simulink model "blance_leg2"  (R2023a)
settings: Solver=VariableStepAuto  StartTime=0.0  StopTime=10  MaxStep=0.0050000000000000001  RelTol=5.0000000000000002e-05  AbsTol=9.9999999999999995e-07
InitFcn:
  | addpath(fileparts(get_param(bdroot,'FileName')));
  | apply_config(bdroot);
model workspace (MAT data in the model file):
  L_length_ref : timeseries (value not decoded)
  L_v_ref : timeseries (value not decoded)
  R_length_ref : timeseries (value not decoded)
  R_v_ref : timeseries (value not decoded)
  runScenario_cfg_override = []
  wheel_speed_compensation = 1
values from neighbouring files (symbols this model uses):
  K = cachedK    [configured_lqr_gain.m]    (also in get_k_length.m = lqr(A,B,Q,R); matlab.mat = [-1.73670717704  -0.157075032659  -0.691811333866  -0.787613)
  N = NM + mp*diff(x + L*sin(theta),t,2)    [get_k_length.m]
  s = sin(phi3 - phi2)    [five_bar_geometry_rm.m]
undefined symbols (not defined in the file or in its folder): X, Y, Z
libraries: sm_lib x82, nesl_utility x35, slpidlib x2
(part 3 of 3)

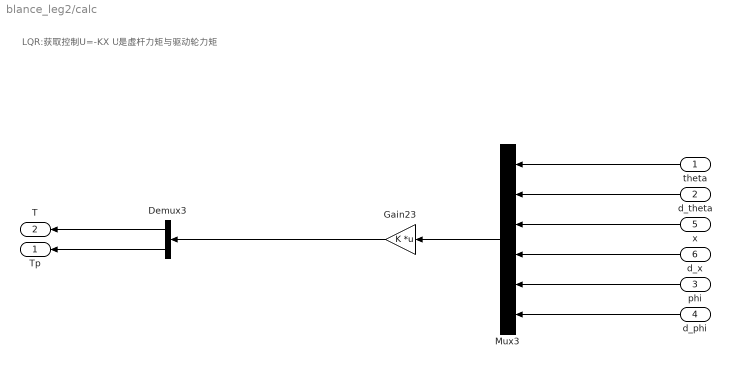
== system blance_leg2/calc ==
  note: LQR:获取控制U=-KX
      | U是虚杆力矩与驱动轮力矩
  theta : Inport
  d_theta : Inport  Port=2
  phi : Inport  Port=3
  d_phi : Inport  Port=4
  x : Inport  Port=5
  d_x : Inport  Port=6
  Demux3 : Demux  Outputs=2
  Gain23 : Gain  Gain=K  Multiplication=Matrix(K*u) (u vector)
  Mux3 : Mux  Inputs=6
  Tp : Outport
  T : Outport  Port=2
  wires:
  Demux3/1 -> T/1
  Demux3/2 -> Tp/1
  Mux3/1 -> Gain23/1
  theta/1 -> Mux3/1
  d_theta/1 -> Mux3/2
  x/1 -> Mux3/3
  d_x/1 -> Mux3/4
  phi/1 -> Mux3/5
  d_phi/1 -> Mux3/6
  Gain23/1 -> Demux3/1

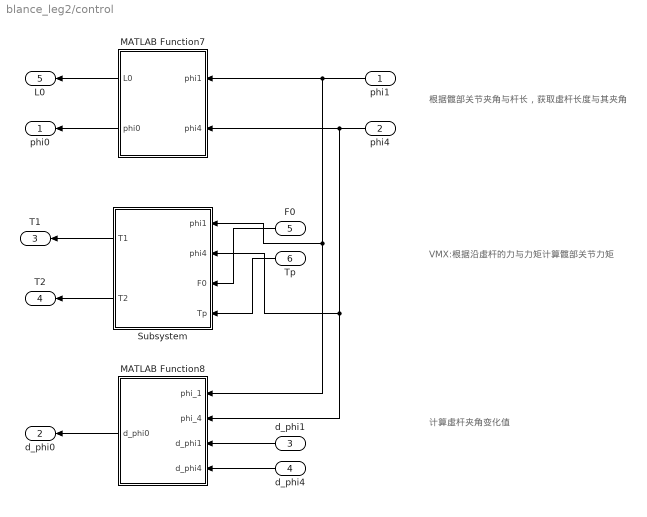
== system blance_leg2/control ==
  note: 计算虚杆夹角变化值
  note: VMX:根据沿虚杆的力与力矩计算髋部关节力矩
  note: 根据髋部关节夹角与杆长，获取虚杆长度与其夹角
  phi1 : Inport
  phi4 : Inport  Port=2
  d_phi1 : Inport  Port=3
  d_phi4 : Inport  Port=4
  F0 : Inport  Port=5
  Tp : Inport  Port=6
  MATLAB Function7 : MATLAB Function  TreatAsAtomicUnit=on
  MATLAB Function8 : MATLAB Function  TreatAsAtomicUnit=on
  Subsystem : Subsystem
  phi0 : Outport
  d_phi0 : Outport  Port=2
  T1 : Outport  Port=3
  T2 : Outport  Port=4
  L0 : Outport  Port=5
  wires:
  MATLAB Function7/2(phi0) -> phi0/1
  MATLAB Function8/1(d_phi0) -> d_phi0/1
  d_phi4/1 -> MATLAB Function8/4(d_phi4)
  d_phi1/1 -> MATLAB Function8/3(d_phi1)
  MATLAB Function7/1(L0) -> L0/1
  phi4/1 -> MATLAB Function7/2(phi4), Subsystem/2(phi4), MATLAB Function8/2(phi_4)
  phi1/1 -> MATLAB Function7/1(phi1), MATLAB Function8/1(phi_1), Subsystem/1(phi1)
  F0/1 -> Subsystem/3(F0)
  Tp/1 -> Subsystem/4(Tp)
  Subsystem/1(T1) -> T1/1
  Subsystem/2(T2) -> T2/1

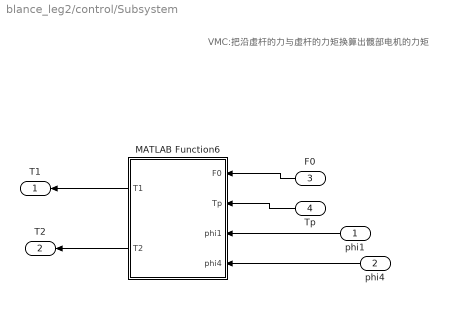
== system blance_leg2/control/Subsystem ==
  note: VMC:把沿虚杆的力与虚杆的力矩换算出髋部电机的力矩
  phi1 : Inport
  phi4 : Inport  Port=2
  F0 : Inport  Port=3
  Tp : Inport  Port=4
  MATLAB Function6 : MATLAB Function  TreatAsAtomicUnit=on
  T1 : Outport
  T2 : Outport  Port=2
  wires:
  phi1/1 -> MATLAB Function6/3(phi1)
  phi4/1 -> MATLAB Function6/4(phi4)
  Tp/1 -> MATLAB Function6/2(Tp)
  MATLAB Function6/1(T1) -> T1/1
  F0/1 -> MATLAB Function6/1(F0)
  MATLAB Function6/2(T2) -> T2/1

== matlab function blance_leg2/Right Wheel Carrier Rate ==
  data: phi1 input; omega output; phi4 input; w1 input; w4 input; bodyPitchRate input
function omega = carrier_world_rate(phi1,phi4,w1,w4,bodyPitchRate)
%#codegen
omega=wheel_carrier_rate(phi1,phi4,w1,w4,bodyPitchRate);
end

== matlab function blance_leg2/Left Wheel Carrier Rate ==
  data: phi1 input; omega output; phi4 input; w1 input; w4 input; bodyPitchRate input
function omega = carrier_world_rate(phi1,phi4,w1,w4,bodyPitchRate)
%#codegen
omega=wheel_carrier_rate(phi1,phi4,w1,w4,bodyPitchRate);
end

== matlab function blance_leg2/Subsystem4/MATLAB Function10 ==
  data: L0 output; phi1 input; phi4 input; phi0 output
function [L0,phi0] = fcn(phi1,phi4)
   
    l5=0.08;%AE长度
    l1=0.075;
    l2=0.14;
    l3=0.14;
    l4=0.075;
    
    YD = l4*sin(phi4);
    YB = l1*sin(phi1);
    XD = l5 + l4*cos(phi4);
    XB = l1*cos(phi1); 
    lBD = sqrt((XD - XB)*(XD - XB) + (YD - YB)*(YD - YB));
    A0 = 2*l2*(XD - XB);
    B0 = 2*l2*(YD - YB);
    C0 = l2*l2 + lBD*lBD - l3*l3;
    phi2 = 2*atan2((B0 + sqrt(A0*A0 + B0*B0 - C0*C0)),(A0 + C0));
    XC = l1*cos(phi1) + l2*cos(phi2);
    YC = l1*sin(phi1) + l2*sin(phi2);
    L0 = sqrt((XC - l5/2)*(XC - l5/2) + YC*YC);
    phi0=atan2(YC,(XC-l5/2));
    
end

== matlab function blance_leg2/Subsystem4/MATLAB Function11 ==
  data: d_phi0 output; phi_1 input; phi_4 input; d_phi1 input; d_phi4 input
function d_phi0 = fcn(phi_1,phi_4,d_phi1,d_phi4)
   
    l5=0.08;%AE长度
    l1=0.075;
    l2=0.14;
    l3=0.14;
    l4=0.075;
    
    d_phi0 = (d_phi1*((l1*cos(phi_1) + (2*l2*cos(2*atan(((4*l2^2*(l1*sin(phi_1) - l4*sin(phi_4))^2 - ((l1*sin(phi_1) - l4*sin(phi_4))^2 + (l5 - l1*cos(phi_1) + l4*cos(phi_4))^2 + l2^2 - l3^2)^2 + 4*l2^2*(l5 - l1*cos(phi_1) + l4*cos(phi_4))^2)^(1/2) - 2*l2*(l1*sin(phi_1) - l4*sin(phi_4)))/((l1*sin(phi_1) - l4*sin(phi_4))^2 + (l5 - l1*cos(phi_1) + l4*cos(phi_4))^2 + l2^2 - l3^2 + 2*l2*(l5 - l1*cos(phi_1) + l4*cos(phi_4)))))*(((8*l1*l2^2*cos(phi_1)*(l1*sin(phi_1) - l4*sin(phi_4)) - 2*(2*l1*cos(phi_1)*(l1*sin(phi_1) - l4*sin(phi_4)) + 2*l1*sin(phi_1)*(l5 - l1*cos(phi_1) + l4*cos(phi_4)))*((l1*sin(phi_1) - l4*sin(phi_4))^2 + (l5 - l1*cos(phi_1) + l4*cos(phi_4))^2 + l2^2 - l3^2) + 8*l1*l2^2*sin(phi_1)*(l5 - l1*cos(phi_1) + l4*cos(phi_4)))/(2*(4*l2^2*(l1*sin(phi_1) - l4*sin(phi_4))^2 - ((l1*sin(phi_1) - l4*sin(phi_4))^2 + (l5 - l1*cos(phi_1) + l4*cos(phi_4))^2 + l2^2 - l3^2)^2 + 4*l2^2*(l5 - l1*cos(phi_1) + l4*cos(phi_4))^2)^(1/2)) - 2*l1*l2*cos(phi_1))/((l1*sin(phi_1) - l4*sin(phi_4))^2 + (l5 - l1*cos(phi_1) + l4*cos(phi_4))^2 + l2^2 - l3^2 + 2*l2*(l5 - l1*cos(phi_1) + l4*cos(phi_4))) - (((4*l2^2*(l1*sin(phi_1) - l4*sin(phi_4))^2 - ((l1*sin(phi_1) - l4*sin(phi_4))^2 + (l5 - l1*cos(phi_1) + l4*cos(phi_4))^2 + l2^2 - l3^2)^2 + 4*l2^2*(l5 - l1*cos(phi_1) + l4*cos(phi_4))^2)^(1/2) - 2*l2*(l1*sin(phi_1) - l4*sin(phi_4)))*(2*l1*l2*sin(phi_1) + 2*l1*cos(phi_1)*(l1*sin(phi_1) - l4*sin(phi_4)) + 2*l1*sin(phi_1)*(l5 - l1*cos(phi_1) + l4*cos(phi_4))))/((l1*sin(phi_1) - l4*sin(phi_4))^2 + (l5 - l1*cos(phi_1) + l4*cos(phi_4))^2 + l2^2 - l3^2 + 2*l2*(l5 - l1*cos(phi_1) + l4*cos(phi_4)))^2))/(((4*l2^2*(l1*sin(phi_1) - l4*sin(phi_4))^2 - ((l1*sin(phi_1) - l4*sin(phi_4))^2 + (l5 - l1*cos(phi_1) + l4*cos(phi_4))^2 + l2^2 - l3^2)^2 + 4*l2^2*(l5 - l1*cos(phi_1) + l4*cos(phi_4))^2)^(1/2) - 2*l2*(l1*sin(phi_1) - l4*sin(phi_4)))^2/((l1*sin(phi_1) - l4*sin(phi_4))^2 + (l5 - l1*cos(phi_1) + l4*cos(phi_4))^2 + l2^2 - l3^2 + 2*l2*(l5 - l1*cos(phi_1) + l4*cos(phi_4)))^2 + 1))/(l2*cos(2*atan(((4*l2^2*(l1*sin(phi_1) - l4*sin(phi_4))^2 - ((l1*sin(phi_1) - l4*sin(phi_4))^2 + (l5 - l1*cos(phi_1) + l4*cos(phi_4))^2 + l2^2 - l3^2)^2 + 4*l2^2*(l5 - l1*cos(phi_1) + l4*cos(phi_4))^2)^(1/2) - 2*l2*(l1*sin(phi_1) - l4*sin(phi_4)))/((l1*sin(phi_1) - l4*sin(phi_4))^2 + (l5 - l1*cos(phi_1) + l4*cos(phi_4))^2 + l2^2 - l3^2 + 2*l2*(l5 - l1*cos(phi_1) + l4*cos(phi_4))))) - l5/2 + l1*cos(phi_1)) + ((l2*sin(2*atan(((4*l2^2*(l1*sin(phi_1) - l4*sin(phi_4))^2 - ((l1*sin(phi_1) - l4*sin(phi_4))^2 + (l5 - l1*cos(phi_1) + l4*cos(phi_4))^2 + l2^2 - l3^2)^2 + 4*l2^2*(l5 - l1*cos(phi_1) + l4*cos(phi_4))^2)^(1/2) - 2*l2*(l1*sin(phi_1) - l4*sin(phi_4)))/((l1*sin(phi_1) - l4*sin(phi_4))^2 + (l5 - l1*cos(phi_1) + l4*cos(phi_4))^2 + l2^2 - l3^2 + 2*l2*(l5 - l1*cos(phi_1) + l4*cos(phi_4))))) + l1*sin(phi_1))*(l1*sin(phi_1) + (2*l2*sin(2*atan(((4*l2^2*(l1*sin(phi_1) - l4*sin(phi_4))^2 - ((l1*sin(phi_1) - l4*sin(phi_4))^2 + (l5 - l1*cos(phi_1) + l4*cos(phi_4))^2 + l2^2 - l3^2)^2 + 4*l2^2*(l5 - l1*cos(phi_1) + l4*cos(phi_4))^2)^(1/2) - 2*l2*(l1*sin(phi_1) - l4*sin(phi_4)))/((l1*sin(phi_1) - l4*sin(phi_4))^2 + (l5 - l1*cos(phi_1) + l4*cos(phi_4))^2 + l2^2 - l3^2 + 2*l2*(l5 - l1*cos(phi_1) + l4*cos(phi_4)))))*(((8*l1*l2^2*cos(phi_1)*(l1*sin(phi_1) - l4*sin(phi_4)) - 2*(2*l1*cos(phi_1)*(l1*sin(phi_1) - l4*sin(phi_4)) + 2*l1*sin(phi_1)*(l5 - l1*cos(phi_1) + l4*cos(phi_4)))*((l1*sin(phi_1) - l4*sin(phi_4))^2 + (l5 - l1*cos(phi_1) + l4*cos(phi_4))^2 + l2^2 - l3^2) + 8*l1*l2^2*sin(phi_1)*(l5 - l1*cos(phi_1) + l4*cos(phi_4)))/(2*(4*l2^2*(l1*sin(phi_1) - l4*sin(phi_4))^2 - ((l1*sin(phi_1) - l4*sin(phi_4))^2 + (l5 - l1*cos(phi_1) + l4*cos(phi_4))^2 + l2^2 - l3^2)^2 + 4*l2^2*(l5 - l1*cos(phi_1) + l4*cos(phi_4))^2)^(1/2)) - 2*l1*l2*cos(phi_1))/((l1*sin(phi_1) - l4*sin(phi_4))^2 + (l5 - l1*cos(phi_1) + l4*cos(phi_4))^2 + l2^2 - l3^2 + 2*l2*(l5 - l1*cos(phi_1) + l4*cos(phi_4))) - (((4*l2^2*(l1*sin(phi_1) - l4*sin(phi_4))^2 - ((l1*sin(phi_1) - l4*sin(phi_4))^2 + (l5 - l1*cos(phi_1) + l4*cos(phi_4))^2 + l2^2 - l3^2)^2 + 4*l2^2*(l5 - l1*cos(phi_1) + l4*cos(phi_4))^2)^(1/2) - 2*l2*(l1*sin(phi_1) - l4*sin(phi_4)))*(2*l1*l2*sin(phi_1) + 2*l1*cos(phi_1)*(l1*sin(phi_1) - l4*sin(phi_4)) + 2*l1*sin(phi_1)*(l5 - l1*cos(phi_1) + l4*cos(phi_4))))/((l1*sin(phi_1) - l4*sin(phi_4))^2 + (l5 - l1*cos(phi_1) + l4*cos(phi_4))^2 + l2^2 - l3^2 + 2*l2*(l5 - l1*cos(phi_1) + l4*cos(phi_4)))^2))/(((4*l2^2*(l1*sin(phi_1) - l4*sin(phi_4))^2 - ((l1*sin(phi_1) - l4*sin(phi_4))^2 + (l5 - l1*cos(phi_1) + l4*cos(phi_4))^2 + l2^2 - l3^2)^2 + 4*l2^2*(l5 - l1*cos(phi_1) + l4*cos(phi_4))^2)^(1/2) - 2*l2*(l1*sin(phi_1) - l4*sin(phi_4)))^2/((l1*sin(phi_1) - l4*sin(phi_4))^2 + (l5 - l1*cos(phi_1) + l4*cos(phi_4))^2 + l2^2 - l3^2 + 2*l2*(l5 - l1*cos(phi_1) + l4*cos(phi_4)))^2 + 1)))/(l2*cos(2*atan(((4*l2^2*(l1*sin(phi_1) - l4*sin(phi_4))^2 - ((l1*sin(phi_1) - l4*sin(phi_4))^2 + (l5 - l1*cos(phi_1) + l4*cos(phi_4))^2 + l2^2 - l3^2)^2 + 4*l2^2*(l5 - l1*cos(phi_1) + l4*cos(phi_4))^2)^(1/2) - 2*l2*(l1*sin(phi_1) - l4*sin(phi_4)))/((l1*sin(phi_1) - l4*sin(phi_4))^2 + (l5 - l1*cos(phi_1) + l4*cos(phi_4))^2 + l2^2 - l3^2 + 2*l2*(l5 - l1*cos(phi_1) + l4*cos(phi_4))))) - l5/2 + l1*cos(phi_1))^2))/((l2*sin(2*atan(((4*l2^2*(l1*sin(phi_1) - l4*sin(phi_4))^2 - ((l1*sin(phi_1) - l4*sin(phi_4))^2 + (l5 - l1*cos(phi_1) + l4*cos(phi_4))^2 + l2^2 - l3^2)^2 + 4*l2^2*(l5 - l1*cos(phi_1) + l4*cos(phi_4))^2)^(1/2) - 2*l2*(l1*sin(phi_1) - l4*sin(phi_4)))/((l1*sin(phi_1) - l4*sin(phi_4))^2 + (l5 - l1*cos(phi_1) + l4*cos(phi_4))^2 + l2^2 - l3^2 + 2*l2*(l5 - l1*cos(phi_1) + l4*cos(phi_4))))) + l1*sin(phi_1))^2/(l2*cos(2*atan(((4*l2^2*(l1*sin(phi_1) - l4*sin(phi_4))^2 - ((l1*sin(phi_1) - l4*sin(phi_4))^2 + (l5 - l1*cos(phi_1) + l4*cos(phi_4))^2 + l2^2 - l3^2)^2 + 4*l2^2*(l5 - l1*cos(phi_1) + l4*cos(phi_4))^2)^(1/2) - 2*l2*(l1*sin(phi_1) - l4*sin(phi_4)))/((l1*sin(phi_1) - l4*sin(phi_4))^2 + (l5 - l1*cos(phi_1) + l4*cos(phi_4))^2 + l2^2 - l3^2 + 2*l2*(l5 - l1*cos(phi_1) + l4*cos(phi_4))))) - l5/2 + l1*cos(phi_1))^2 + 1) - (d_phi4*((2*l2*cos(2*atan(((4*l2^2*(l1*sin(phi_1) - l4*sin(phi_4))^2 - ((l1*sin(phi_1) - l4*sin(phi_4))^2 + (l5 - l1*cos(phi_1) + l4*cos(phi_4))^2 + l2^2 - l3^2)^2 + 4*l2^2*(l5 - l1*cos(phi_1) + l4*cos(phi_4))^2)^(1/2) - 2*l2*(l1*sin(phi_1) - l4*sin(phi_4)))/((l1*sin(phi_1) - l4*sin(phi_4))^2 + (l5 - l1*cos(phi_1) + l4*cos(phi_4))^2 + l2^2 - l3^2 + 2*l2*(l5 - l1*cos(phi_1) + l4*cos(phi_4)))))*(((8*l2^2*l4*cos(phi_4)*(l1*sin(phi_1) - l4*sin(phi_4)) - 2*(2*l4*cos(phi_4)*(l1*sin(phi_1) - l4*sin(phi_4)) + 2*l4*sin(phi_4)*(l5 - l1*cos(phi_1) + l4*cos(phi_4)))*((l1*sin(phi_1) - l4*sin(phi_4))^2 + (l5 - l1*cos(phi_1) + l4*cos(phi_4))^2 + l2^2 - l3^2) + 8*l2^2*l4*sin(phi_4)*(l5 - l1*cos(phi_1) + l4*cos(phi_4)))/(2*(4*l2^2*(l1*sin(phi_1) - l4*sin(phi_4))^2 - ((l1*sin(phi_1) - l4*sin(phi_4))^2 + (l5 - l1*cos(phi_1) + l4*cos(phi_4))^2 + l2^2 - l3^2)^2 + 4*l2^2*(l5 - l1*cos(phi_1) + l4*cos(phi_4))^2)^(1/2)) - 2*l2*l4*cos(phi_4))/((l1*sin(phi_1) - l4*sin(phi_4))^2 + (l5 - l1*cos(phi_1) + l4*cos(phi_4))^2 + l2^2 - l3^2 + 2*l2*(l5 - l1*cos(phi_1) + l4*cos(phi_4))) - (((4*l2^2*(l1*sin(phi_1) - l4*sin(phi_4))^2 - ((l1*sin(phi_1) - l4*sin(phi_4))^2 + (l5 - l1*cos(phi_1) + l4*cos(phi_4))^2 + l2^2 - l3^2)^2 + 4*l2^2*(l5 - l1*cos(phi_1) + l4*cos(phi_4))^2)^(1/2) - 2*l2*(l1*sin(phi_1) - l4*sin(phi_4)))*(2*l2*l4*sin(phi_4) + 2*l4*cos(phi_4)*(l1*sin(phi_1) - l4*sin(phi_4)) + 2*l4*sin(phi_4)*(l5 - l1*cos(phi_1) + l4*cos(phi_4))))/((l1*sin(phi_1) - l4*sin(phi_4))^2 + (l5 - l1*cos(phi_1) + l4*cos(phi_4))^2 + l2^2 - l3^2 + 2*l2*(l5 - l1*cos(phi_1) + l4*cos(phi_4)))^2))/((((4*l2^2*(l1*sin(phi_1) - l4*sin(phi_4))^2 - ((l1*sin(phi_1) - l4*sin(phi_4))^2 + (l5 - l1*cos(phi_1) + l4*cos(phi_4))^2 + l2^2 - l3^2)^2 + 4*l2^2*(l5 - l1*cos(phi_1) + l4*cos(phi_4))^2)^(1/2) - 2*l2*(l1*sin(phi_1) - l4*sin(phi_4)))^2/((l1*sin(phi_1) - l4*sin(phi_4))^2 + (l5 - l1*cos(phi_1) + l4*cos(phi_4))^2 + l2^2 - l3^2 + 2*l2*(l5 - l1*cos(phi_1) + l4*cos(phi_4)))^2 + 1)*(l2*cos(2*atan(((4*l2^2*(l1*sin(phi_1) - l4*sin(phi_4))^2 - ((l1*sin(phi_1) - l4*sin(phi_4))^2 + (l5 - l1*cos(phi_1) + l4*cos(phi_4))^2 + l2^2 - l3^2)^2 + 4*l2^2*(l5 - l1*cos(phi_1) + l4*cos(phi_4))^2)^(1/2) - 2*l2*(l1*sin(phi_1) - l4*sin(phi_4)))/((l1*sin(phi_1) - l4*sin(phi_4))^2 + (l5 - l1*cos(phi_1) + l4*cos(phi_4))^2 + l2^2 - l3^2 + 2*l2*(l5 - l1*cos(phi_1) + l4*cos(phi_4))))) - l5/2 + l1*cos(phi_1))) + (2*l2*sin(2*atan(((4*l2^2*(l1*sin(phi_1) - l4*sin(phi_4))^2 - ((l1*sin(phi_1) - l4*sin(phi_4))^2 + (l5 - l1*cos(phi_1) + l4*cos(phi_4))^2 + l2^2 - l3^2)^2 + 4*l2^2*(l5 - l1*cos(phi_1) + l4*cos(phi_4))^2)^(1/2) - 2*l2*(l1*sin(phi_1) - l4*sin(phi_4)))/((l1*sin(phi_1) - l4*sin(phi_4))^2 + (l5 - l1*cos(phi_1) + l4*cos(phi_4))^2 + l2^2 - l3^2 + 2*l2*(l5 - l1*cos(phi_1) + l4*cos(phi_4)))))*(l2*sin(2*atan(((4*l2^2*(l1*sin(phi_1) - l4*sin(phi_4))^2 - ((l1*sin(phi_1) - l4*sin(phi_4))^2 + (l5 - l1*cos(phi_1) + l4*cos(phi_4))^2 + l2^2 - l3^2)^2 + 4*l2^2*(l5 - l1*cos(phi_1) + l4*cos(phi_4))^2)^(1/2) - 2*l2*(l1*sin(phi_1) - l4*sin(phi_4)))/((l1*sin(phi_1) - l4*sin(phi_4))^2 + (l5 - l1*cos(phi_1) + l4*cos(phi_4))^2 + l2^2 - l3^2 + 2*l2*(l5 - l1*cos(phi_1) + l4*cos(phi_4))))) + l1*sin(phi_1))*(((8*l2^2*l4*cos(phi_4)*(l1*sin(phi_1) - l4*sin(phi_4)) - 2*(2*l4*cos(phi_4)*(l1*sin(phi_1) - l4*sin(phi_4)) + 2*l4*sin(phi_4)*(l5 - l1*cos(phi_1) + l4*cos(phi_4)))*((l1*sin(phi_1) - l4*sin(phi_4))^2 + (l5 - l1*cos(phi_1) + l4*cos(phi_4))^2 + l2^2 - l3^2) + 8*l2^2*l4*sin(phi_4)*(l5 - l1*cos(phi_1) + l4*cos(phi_4)))/(2*(4*l2^2*(l1*sin(phi_1) - l4*sin(phi_4))^2 - ((l1*sin(phi_1) - l4*sin(phi_4))^2 + (l5 - l1*cos(phi_1) + l4*cos(phi_4))^2 + l2^2 - l3^2)^2 + 4*l2^2*(l5 - l1*cos(phi_1) + l4*cos(phi_4))^2)^(1/2)) - 2*l2*l4*cos(phi_4))/((l1*sin(phi_1) - l4*sin(phi_4))^2 + (l5 - l1*cos(phi_1) + l4*cos(phi_4))^2 + l2^2 - l3^2 + 2*l2*(l5 - l1*cos(phi_1) + l4*cos(phi_4))) - (((4*l2^2*(l1*sin(phi_1) - l4*sin(phi_4))^2 - ((l1*sin(phi_1) - l4*sin(phi_4))^2 + (l5 - l1*cos(phi_1) + l4*cos(phi_4))^2 + l2^2 - l3^2)^2 + 4*l2^2*(l5 - l1*cos(phi_1) + l4*cos(phi_4))^2)^(1/2) - 2*l2*(l1*sin(phi_1) - l4*sin(phi_4)))*(2*l2*l4*sin(phi_4) + 2*l4*cos(phi_4)*(l1*sin(phi_1) - l4*sin(phi_4)) + 2*l4*sin(phi_4)*(l5 - l1*cos(phi_1) + l4*cos(phi_4))))/((l1*sin(phi_1) - l4*sin(phi_4))^2 + (l5 - l1*cos(phi_1) + l4*cos(phi_4))^2 + l2^2 - l3^2 + 2*l2*(l5 - l1*cos(phi_1) + l4*cos(phi_4)))^2))/((((4*l2^2*(l1*sin(phi_1) - l4*sin(phi_4))^2 - ((l1*sin(phi_1) - l4*sin(phi_4))^2 + (l5 - l1*cos(phi_1) + l4*cos(phi_4))^2 + l2^2 - l3^2)^2 + 4*l2^2*(l5 - l1*cos(phi_1) + l4*cos(phi_4))^2)^(1/2) - 2*l2*(l1*sin(phi_1) - l4*sin(phi_4)))^2/((l1*sin(phi_1) - l4*sin(phi_4))^2 + (l5 - l1*cos(phi_1) + l4*cos(phi_4))^2 + l2^2 - l3^2 + 2*l2*(l5 - l1*cos(phi_1) + l4*cos(phi_4)))^2 + 1)*(l2*cos(2*atan(((4*l2^2*(l1*sin(phi_1) - l4*sin(phi_4))^2 - ((l1*sin(phi_1) - l4*sin(phi_4))^2 + (l5 - l1*cos(phi_1) + l4*cos(phi_4))^2 + l2^2 - l3^2)^2 + 4*l2^2*(l5 - l1*cos(phi_1) + l4*cos(phi_4))^2)^(1/2) - 2*l2*(l1*sin(phi_1) - l4*sin(phi_4)))/((l1*sin(phi_1) - l4*sin(phi_4))^2 + (l5 - l1*cos(phi_1) + l4*cos(phi_4))^2 + l2^2 - l3^2 + 2*l2*(l5 - l1*cos(phi_1) + l4*cos(phi_4))))) - l5/2 + l1*cos(phi_1))^2)))/((l2*sin(2*atan(((4*l2^2*(l1*sin(phi_1) - l4*sin(phi_4))^2 - ((l1*sin(phi_1) - l4*sin(phi_4))^2 + (l5 - l1*cos(phi_1) + l4*cos(phi_4))^2 + l2^2 - l3^2)^2 + 4*l2^2*(l5 - l1*cos(phi_1) + l4*cos(phi_4))^2)^(1/2) - 2*l2*(l1*sin(phi_1) - l4*sin(phi_4)))/((l1*sin(phi_1) - l4*sin(phi_4))^2 + (l5 - l1*cos(phi_1) + l4*cos(phi_4))^2 + l2^2 - l3^2 + 2*l2*(l5 - l1*cos(phi_1) + l4*cos(phi_4))))) + l1*sin(phi_1))^2/(l2*cos(2*atan(((4*l2^2*(l1*sin(phi_1) - l4*sin(phi_4))^2 - ((l1*sin(phi_1) - l4*sin(phi_4))^2 + (l5 - l1*cos(phi_1) + l4*cos(phi_4))^2 + l2^2 - l3^2)^2 + 4*l2^2*(l5 - l1*cos(phi_1) + l4*cos(phi_4))^2)^(1/2) - 2*l2*(l1*sin(phi_1) - l4*sin(phi_4)))/((l1*sin(phi_1) - l4*sin(phi_4))^2 + (l5 - l1*cos(phi_1) + l4*cos(phi_4))^2 + l2^2 - l3^2 + 2*l2*(l5 - l1*cos(phi_1) + l4*cos(phi_4))))) - l5/2 + l1*cos(phi_1))^2 + 1);
end
    % syms phi_0 phi_1 phi_2 phi_4 l1 l2 l3 l4 l5 L0 d_phi1 d_phi4
    % 
    % XD=l5+l4*cos(phi_4);
    % YD=l4*sin(phi_4);
    % XB=l1*cos(phi_1);
    % YB=l1*sin(phi_1);
    % A0=2*l2*(XD-XB);
    % B0=2*l2*(YD-YB);
    % lBD=sqrt((XD-XB)^2+(YD-YB)^2);
    % C0=l2^2+lBD^2-l3^2;
    % phi_2=2*atan((B0+sqrt(A0^2+B0^2-C0^2))/(A0+C0));
    % XC=XB+l2*cos(phi_2);
    % YC=YB+l2*sin(phi_2);
    % L0=sqrt((XC-l5/2)^2+YC^2);
    % phi_0=atan(YC/(XC-l5/2));
    % 
    % J=jacobian([L0;phi_0],[phi_1;phi_4]);
    % phi0_dot = J(2,1)*d_phi1 +J(2,2)*d_phi4

    % jacobian函数无法在simulink中使用，故直接使用jacobian函数的最终结果

== matlab function blance_leg2/control/Subsystem/MATLAB Function6 ==
  data: F0 input; T1 output; Tp input; phi1 input; phi4 input; T2 output
function [T1,T2] = VMC_calc(F0,Tp,phi1,phi4)

    l5=0.08;%AE长度
    l1=0.075;
    l2=0.14;
    l3=0.14;
    l4=0.075;

YD = l4*sin(phi4);
YB = l1*sin(phi1);
XD = l5 + l4*cos(phi4);
XB = l1*cos(phi1); 
lBD = sqrt((XD - XB)*(XD - XB) + (YD - YB)*(YD - YB));
A0 = 2*l2*(XD - XB);
B0 = 2*l2*(YD - YB);
C0 = l2*l2 + lBD*lBD - l3*l3;
phi2 = 2*atan2((B0 + sqrt(A0*A0 + B0*B0 - C0*C0)),A0 + C0);
phi3 = atan2(YB-YD+l2*sin(phi2),XB-XD+l2*cos(phi2));
XC = l1*cos(phi1) + l2*cos(phi2);
YC = l1*sin(phi1) + l2*sin(phi2);
L0 = sqrt((XC - l5/2)*(XC - l5/2) + YC*YC);
phi0 = atan2(YC,XC - l5/2);
j11 = (l1*sin(phi0-phi3)*sin(phi1-phi2))/sin(phi3-phi2);
j12 = (l1*cos(phi0-phi3)*sin(phi1-phi2))/(L0*sin(phi3-phi2));
j21 = (l4*sin(phi0-phi2)*sin(phi3-phi4))/sin(phi3-phi2);
j22 = (l4*cos(phi0-phi2)*sin(phi3-phi4))/(L0*sin(phi3-phi2));
J = [j11 j12; j21 j22];
F = [F0;Tp];
T = J * F;
T1 = T(1,1);
T2 = T(2,1);

end

== matlab function blance_leg2/control/MATLAB Function7 ==
  data: L0 output; phi1 input; phi4 input; phi0 output
function [L0,phi0] = fcn(phi1,phi4)
  
    l5=0.08;%AE长度
    l1=0.075;
    l2=0.14;
    l3=0.14;
    l4=0.075;
    
    YD = l4*sin(phi4);
    YB = l1*sin(phi1);
    XD = l5 + l4*cos(phi4);
    XB = l1*cos(phi1); 
    lBD = sqrt((XD - XB)*(XD - XB) + (YD - YB)*(YD - YB));
    A0 = 2*l2*(XD - XB);
    B0 = 2*l2*(YD - YB);
    C0 = l2*l2 + lBD*lBD - l3*l3;
    phi2 = 2*atan2((B0 + sqrt(A0*A0 + B0*B0 - C0*C0)),(A0 + C0));
    XC = l1*cos(phi1) + l2*cos(phi2);
    YC = l1*sin(phi1) + l2*sin(phi2);
    L0 = sqrt((XC - l5/2)*(XC - l5/2) + YC*YC);
    phi0=atan2(YC,(XC-l5/2));
end

== matlab function blance_leg2/control/MATLAB Function8 ==
  data: d_phi0 output; phi_1 input; phi_4 input; d_phi1 input; d_phi4 input
% 计算虚杆夹角变化值
function d_phi0 = fcn(phi_1,phi_4,d_phi1,d_phi4)
   
    l5=0.08;%AE长度
    l1=0.075;
    l2=0.14;
    l3=0.14;
    l4=0.075;
    
    d_phi0 = (d_phi1*((l1*cos(phi_1) + (2*l2*cos(2*atan(((4*l2^2*(l1*sin(phi_1) - l4*sin(phi_4))^2 - ((l1*sin(phi_1) - l4*sin(phi_4))^2 + (l5 - l1*cos(phi_1) + l4*cos(phi_4))^2 + l2^2 - l3^2)^2 + 4*l2^2*(l5 - l1*cos(phi_1) + l4*cos(phi_4))^2)^(1/2) - 2*l2*(l1*sin(phi_1) - l4*sin(phi_4)))/((l1*sin(phi_1) - l4*sin(phi_4))^2 + (l5 - l1*cos(phi_1) + l4*cos(phi_4))^2 + l2^2 - l3^2 + 2*l2*(l5 - l1*cos(phi_1) + l4*cos(phi_4)))))*(((8*l1*l2^2*cos(phi_1)*(l1*sin(phi_1) - l4*sin(phi_4)) - 2*(2*l1*cos(phi_1)*(l1*sin(phi_1) - l4*sin(phi_4)) + 2*l1*sin(phi_1)*(l5 - l1*cos(phi_1) + l4*cos(phi_4)))*((l1*sin(phi_1) - l4*sin(phi_4))^2 + (l5 - l1*cos(phi_1) + l4*cos(phi_4))^2 + l2^2 - l3^2) + 8*l1*l2^2*sin(phi_1)*(l5 - l1*cos(phi_1) + l4*cos(phi_4)))/(2*(4*l2^2*(l1*sin(phi_1) - l4*sin(phi_4))^2 - ((l1*sin(phi_1) - l4*sin(phi_4))^2 + (l5 - l1*cos(phi_1) + l4*cos(phi_4))^2 + l2^2 - l3^2)^2 + 4*l2^2*(l5 - l1*cos(phi_1) + l4*cos(phi_4))^2)^(1/2)) - 2*l1*l2*cos(phi_1))/((l1*sin(phi_1) - l4*sin(phi_4))^2 + (l5 - l1*cos(phi_1) + l4*cos(phi_4))^2 + l2^2 - l3^2 + 2*l2*(l5 - l1*cos(phi_1) + l4*cos(phi_4))) - (((4*l2^2*(l1*sin(phi_1) - l4*sin(phi_4))^2 - ((l1*sin(phi_1) - l4*sin(phi_4))^2 + (l5 - l1*cos(phi_1) + l4*cos(phi_4))^2 + l2^2 - l3^2)^2 + 4*l2^2*(l5 - l1*cos(phi_1) + l4*cos(phi_4))^2)^(1/2) - 2*l2*(l1*sin(phi_1) - l4*sin(phi_4)))*(2*l1*l2*sin(phi_1) + 2*l1*cos(phi_1)*(l1*sin(phi_1) - l4*sin(phi_4)) + 2*l1*sin(phi_1)*(l5 - l1*cos(phi_1) + l4*cos(phi_4))))/((l1*sin(phi_1) - l4*sin(phi_4))^2 + (l5 - l1*cos(phi_1) + l4*cos(phi_4))^2 + l2^2 - l3^2 + 2*l2*(l5 - l1*cos(phi_1) + l4*cos(phi_4)))^2))/(((4*l2^2*(l1*sin(phi_1) - l4*sin(phi_4))^2 - ((l1*sin(phi_1) - l4*sin(phi_4))^2 + (l5 - l1*cos(phi_1) + l4*cos(phi_4))^2 + l2^2 - l3^2)^2 + 4*l2^2*(l5 - l1*cos(phi_1) + l4*cos(phi_4))^2)^(1/2) - 2*l2*(l1*sin(phi_1) - l4*sin(phi_4)))^2/((l1*sin(phi_1) - l4*sin(phi_4))^2 + (l5 - l1*cos(phi_1) + l4*cos(phi_4))^2 + l2^2 - l3^2 + 2*l2*(l5 - l1*cos(phi_1) + l4*cos(phi_4)))^2 + 1))/(l2*cos(2*atan(((4*l2^2*(l1*sin(phi_1) - l4*sin(phi_4))^2 - ((l1*sin(phi_1) - l4*sin(phi_4))^2 + (l5 - l1*cos(phi_1) + l4*cos(phi_4))^2 + l2^2 - l3^2)^2 + 4*l2^2*(l5 - l1*cos(phi_1) + l4*cos(phi_4))^2)^(1/2) - 2*l2*(l1*sin(phi_1) - l4*sin(phi_4)))/((l1*sin(phi_1) - l4*sin(phi_4))^2 + (l5 - l1*cos(phi_1) + l4*cos(phi_4))^2 + l2^2 - l3^2 + 2*l2*(l5 - l1*cos(phi_1) + l4*cos(phi_4))))) - l5/2 + l1*cos(phi_1)) + ((l2*sin(2*atan(((4*l2^2*(l1*sin(phi_1) - l4*sin(phi_4))^2 - ((l1*sin(phi_1) - l4*sin(phi_4))^2 + (l5 - l1*cos(phi_1) + l4*cos(phi_4))^2 + l2^2 - l3^2)^2 + 4*l2^2*(l5 - l1*cos(phi_1) + l4*cos(phi_4))^2)^(1/2) - 2*l2*(l1*sin(phi_1) - l4*sin(phi_4)))/((l1*sin(phi_1) - l4*sin(phi_4))^2 + (l5 - l1*cos(phi_1) + l4*cos(phi_4))^2 + l2^2 - l3^2 + 2*l2*(l5 - l1*cos(phi_1) + l4*cos(phi_4))))) + l1*sin(phi_1))*(l1*sin(phi_1) + (2*l2*sin(2*atan(((4*l2^2*(l1*sin(phi_1) - l4*sin(phi_4))^2 - ((l1*sin(phi_1) - l4*sin(phi_4))^2 + (l5 - l1*cos(phi_1) + l4*cos(phi_4))^2 + l2^2 - l3^2)^2 + 4*l2^2*(l5 - l1*cos(phi_1) + l4*cos(phi_4))^2)^(1/2) - 2*l2*(l1*sin(phi_1) - l4*sin(phi_4)))/((l1*sin(phi_1) - l4*sin(phi_4))^2 + (l5 - l1*cos(phi_1) + l4*cos(phi_4))^2 + l2^2 - l3^2 + 2*l2*(l5 - l1*cos(phi_1) + l4*cos(phi_4)))))*(((8*l1*l2^2*cos(phi_1)*(l1*sin(phi_1) - l4*sin(phi_4)) - 2*(2*l1*cos(phi_1)*(l1*sin(phi_1) - l4*sin(phi_4)) + 2*l1*sin(phi_1)*(l5 - l1*cos(phi_1) + l4*cos(phi_4)))*((l1*sin(phi_1) - l4*sin(phi_4))^2 + (l5 - l1*cos(phi_1) + l4*cos(phi_4))^2 + l2^2 - l3^2) + 8*l1*l2^2*sin(phi_1)*(l5 - l1*cos(phi_1) + l4*cos(phi_4)))/(2*(4*l2^2*(l1*sin(phi_1) - l4*sin(phi_4))^2 - ((l1*sin(phi_1) - l4*sin(phi_4))^2 + (l5 - l1*cos(phi_1) + l4*cos(phi_4))^2 + l2^2 - l3^2)^2 + 4*l2^2*(l5 - l1*cos(phi_1) + l4*cos(phi_4))^2)^(1/2)) - 2*l1*l2*cos(phi_1))/((l1*sin(phi_1) - l4*sin(phi_4))^2 + (l5 - l1*cos(phi_1) + l4*cos(phi_4))^2 + l2^2 - l3^2 + 2*l2*(l5 - l1*cos(phi_1) + l4*cos(phi_4))) - (((4*l2^2*(l1*sin(phi_1) - l4*sin(phi_4))^2 - ((l1*sin(phi_1) - l4*sin(phi_4))^2 + (l5 - l1*cos(phi_1) + l4*cos(phi_4))^2 + l2^2 - l3^2)^2 + 4*l2^2*(l5 - l1*cos(phi_1) + l4*cos(phi_4))^2)^(1/2) - 2*l2*(l1*sin(phi_1) - l4*sin(phi_4)))*(2*l1*l2*sin(phi_1) + 2*l1*cos(phi_1)*(l1*sin(phi_1) - l4*sin(phi_4)) + 2*l1*sin(phi_1)*(l5 - l1*cos(phi_1) + l4*cos(phi_4))))/((l1*sin(phi_1) - l4*sin(phi_4))^2 + (l5 - l1*cos(phi_1) + l4*cos(phi_4))^2 + l2^2 - l3^2 + 2*l2*(l5 - l1*cos(phi_1) + l4*cos(phi_4)))^2))/(((4*l2^2*(l1*sin(phi_1) - l4*sin(phi_4))^2 - ((l1*sin(phi_1) - l4*sin(phi_4))^2 + (l5 - l1*cos(phi_1) + l4*cos(phi_4))^2 + l2^2 - l3^2)^2 + 4*l2^2*(l5 - l1*cos(phi_1) + l4*cos(phi_4))^2)^(1/2) - 2*l2*(l1*sin(phi_1) - l4*sin(phi_4)))^2/((l1*sin(phi_1) - l4*sin(phi_4))^2 + (l5 - l1*cos(phi_1) + l4*cos(phi_4))^2 + l2^2 - l3^2 + 2*l2*(l5 - l1*cos(phi_1) + l4*cos(phi_4)))^2 + 1)))/(l2*cos(2*atan(((4*l2^2*(l1*sin(phi_1) - l4*sin(phi_4))^2 - ((l1*sin(phi_1) - l4*sin(phi_4))^2 + (l5 - l1*cos(phi_1) + l4*cos(phi_4))^2 + l2^2 - l3^2)^2 + 4*l2^2*(l5 - l1*cos(phi_1) + l4*cos(phi_4))^2)^(1/2) - 2*l2*(l1*sin(phi_1) - l4*sin(phi_4)))/((l1*sin(phi_1) - l4*sin(phi_4))^2 + (l5 - l1*cos(phi_1) + l4*cos(phi_4))^2 + l2^2 - l3^2 + 2*l2*(l5 - l1*cos(phi_1) + l4*cos(phi_4))))) - l5/2 + l1*cos(phi_1))^2))/((l2*sin(2*atan(((4*l2^2*(l1*sin(phi_1) - l4*sin(phi_4))^2 - ((l1*sin(phi_1) - l4*sin(phi_4))^2 + (l5 - l1*cos(phi_1) + l4*cos(phi_4))^2 + l2^2 - l3^2)^2 + 4*l2^2*(l5 - l1*cos(phi_1) + l4*cos(phi_4))^2)^(1/2) - 2*l2*(l1*sin(phi_1) - l4*sin(phi_4)))/((l1*sin(phi_1) - l4*sin(phi_4))^2 + (l5 - l1*cos(phi_1) + l4*cos(phi_4))^2 + l2^2 - l3^2 + 2*l2*(l5 - l1*cos(phi_1) + l4*cos(phi_4))))) + l1*sin(phi_1))^2/(l2*cos(2*atan(((4*l2^2*(l1*sin(phi_1) - l4*sin(phi_4))^2 - ((l1*sin(phi_1) - l4*sin(phi_4))^2 + (l5 - l1*cos(phi_1) + l4*cos(phi_4))^2 + l2^2 - l3^2)^2 + 4*l2^2*(l5 - l1*cos(phi_1) + l4*cos(phi_4))^2)^(1/2) - 2*l2*(l1*sin(phi_1) - l4*sin(phi_4)))/((l1*sin(phi_1) - l4*sin(phi_4))^2 + (l5 - l1*cos(phi_1) + l4*cos(phi_4))^2 + l2^2 - l3^2 + 2*l2*(l5 - l1*cos(phi_1) + l4*cos(phi_4))))) - l5/2 + l1*cos(phi_1))^2 + 1) - (d_phi4*((2*l2*cos(2*atan(((4*l2^2*(l1*sin(phi_1) - l4*sin(phi_4))^2 - ((l1*sin(phi_1) - l4*sin(phi_4))^2 + (l5 - l1*cos(phi_1) + l4*cos(phi_4))^2 + l2^2 - l3^2)^2 + 4*l2^2*(l5 - l1*cos(phi_1) + l4*cos(phi_4))^2)^(1/2) - 2*l2*(l1*sin(phi_1) - l4*sin(phi_4)))/((l1*sin(phi_1) - l4*sin(phi_4))^2 + (l5 - l1*cos(phi_1) + l4*cos(phi_4))^2 + l2^2 - l3^2 + 2*l2*(l5 - l1*cos(phi_1) + l4*cos(phi_4)))))*(((8*l2^2*l4*cos(phi_4)*(l1*sin(phi_1) - l4*sin(phi_4)) - 2*(2*l4*cos(phi_4)*(l1*sin(phi_1) - l4*sin(phi_4)) + 2*l4*sin(phi_4)*(l5 - l1*cos(phi_1) + l4*cos(phi_4)))*((l1*sin(phi_1) - l4*sin(phi_4))^2 + (l5 - l1*cos(phi_1) + l4*cos(phi_4))^2 + l2^2 - l3^2) + 8*l2^2*l4*sin(phi_4)*(l5 - l1*cos(phi_1) + l4*cos(phi_4)))/(2*(4*l2^2*(l1*sin(phi_1) - l4*sin(phi_4))^2 - ((l1*sin(phi_1) - l4*sin(phi_4))^2 + (l5 - l1*cos(phi_1) + l4*cos(phi_4))^2 + l2^2 - l3^2)^2 + 4*l2^2*(l5 - l1*cos(phi_1) + l4*cos(phi_4))^2)^(1/2)) - 2*l2*l4*cos(phi_4))/((l1*sin(phi_1) - l4*sin(phi_4))^2 + (l5 - l1*cos(phi_1) + l4*cos(phi_4))^2 + l2^2 - l3^2 + 2*l2*(l5 - l1*cos(phi_1) + l4*cos(phi_4))) - (((4*l2^2*(l1*sin(phi_1) - l4*sin(phi_4))^2 - ((l1*sin(phi_1) - l4*sin(phi_4))^2 + (l5 - l1*cos(phi_1) + l4*cos(phi_4))^2 + l2^2 - l3^2)^2 + 4*l2^2*(l5 - l1*cos(phi_1) + l4*cos(phi_4))^2)^(1/2) - 2*l2*(l1*sin(phi_1) - l4*sin(phi_4)))*(2*l2*l4*sin(phi_4) + 2*l4*cos(phi_4)*(l1*sin(phi_1) - l4*sin(phi_4)) + 2*l4*sin(phi_4)*(l5 - l1*cos(phi_1) + l4*cos(phi_4))))/((l1*sin(phi_1) - l4*sin(phi_4))^2 + (l5 - l1*cos(phi_1) + l4*cos(phi_4))^2 + l2^2 - l3^2 + 2*l2*(l5 - l1*cos(phi_1) + l4*cos(phi_4)))^2))/((((4*l2^2*(l1*sin(phi_1) - l4*sin(phi_4))^2 - ((l1*sin(phi_1) - l4*sin(phi_4))^2 + (l5 - l1*cos(phi_1) + l4*cos(phi_4))^2 + l2^2 - l3^2)^2 + 4*l2^2*(l5 - l1*cos(phi_1) + l4*cos(phi_4))^2)^(1/2) - 2*l2*(l1*sin(phi_1) - l4*sin(phi_4)))^2/((l1*sin(phi_1) - l4*sin(phi_4))^2 + (l5 - l1*cos(phi_1) + l4*cos(phi_4))^2 + l2^2 - l3^2 + 2*l2*(l5 - l1*cos(phi_1) + l4*cos(phi_4)))^2 + 1)*(l2*cos(2*atan(((4*l2^2*(l1*sin(phi_1) - l4*sin(phi_4))^2 - ((l1*sin(phi_1) - l4*sin(phi_4))^2 + (l5 - l1*cos(phi_1) + l4*cos(phi_4))^2 + l2^2 - l3^2)^2 + 4*l2^2*(l5 - l1*cos(phi_1) + l4*cos(phi_4))^2)^(1/2) - 2*l2*(l1*sin(phi_1) - l4*sin(phi_4)))/((l1*sin(phi_1) - l4*sin(phi_4))^2 + (l5 - l1*cos(phi_1) + l4*cos(phi_4))^2 + l2^2 - l3^2 + 2*l2*(l5 - l1*cos(phi_1) + l4*cos(phi_4))))) - l5/2 + l1*cos(phi_1))) + (2*l2*sin(2*atan(((4*l2^2*(l1*sin(phi_1) - l4*sin(phi_4))^2 - ((l1*sin(phi_1) - l4*sin(phi_4))^2 + (l5 - l1*cos(phi_1) + l4*cos(phi_4))^2 + l2^2 - l3^2)^2 + 4*l2^2*(l5 - l1*cos(phi_1) + l4*cos(phi_4))^2)^(1/2) - 2*l2*(l1*sin(phi_1) - l4*sin(phi_4)))/((l1*sin(phi_1) - l4*sin(phi_4))^2 + (l5 - l1*cos(phi_1) + l4*cos(phi_4))^2 + l2^2 - l3^2 + 2*l2*(l5 - l1*cos(phi_1) + l4*cos(phi_4)))))*(l2*sin(2*atan(((4*l2^2*(l1*sin(phi_1) - l4*sin(phi_4))^2 - ((l1*sin(phi_1) - l4*sin(phi_4))^2 + (l5 - l1*cos(phi_1) + l4*cos(phi_4))^2 + l2^2 - l3^2)^2 + 4*l2^2*(l5 - l1*cos(phi_1) + l4*cos(phi_4))^2)^(1/2) - 2*l2*(l1*sin(phi_1) - l4*sin(phi_4)))/((l1*sin(phi_1) - l4*sin(phi_4))^2 + (l5 - l1*cos(phi_1) + l4*cos(phi_4))^2 + l2^2 - l3^2 + 2*l2*(l5 - l1*cos(phi_1) + l4*cos(phi_4))))) + l1*sin(phi_1))*(((8*l2^2*l4*cos(phi_4)*(l1*sin(phi_1) - l4*sin(phi_4)) - 2*(2*l4*cos(phi_4)*(l1*sin(phi_1) - l4*sin(phi_4)) + 2*l4*sin(phi_4)*(l5 - l1*cos(phi_1) + l4*cos(phi_4)))*((l1*sin(phi_1) - l4*sin(phi_4))^2 + (l5 - l1*cos(phi_1) + l4*cos(phi_4))^2 + l2^2 - l3^2) + 8*l2^2*l4*sin(phi_4)*(l5 - l1*cos(phi_1) + l4*cos(phi_4)))/(2*(4*l2^2*(l1*sin(phi_1) - l4*sin(phi_4))^2 - ((l1*sin(phi_1) - l4*sin(phi_4))^2 + (l5 - l1*cos(phi_1) + l4*cos(phi_4))^2 + l2^2 - l3^2)^2 + 4*l2^2*(l5 - l1*cos(phi_1) + l4*cos(phi_4))^2)^(1/2)) - 2*l2*l4*cos(phi_4))/((l1*sin(phi_1) - l4*sin(phi_4))^2 + (l5 - l1*cos(phi_1) + l4*cos(phi_4))^2 + l2^2 - l3^2 + 2*l2*(l5 - l1*cos(phi_1) + l4*cos(phi_4))) - (((4*l2^2*(l1*sin(phi_1) - l4*sin(phi_4))^2 - ((l1*sin(phi_1) - l4*sin(phi_4))^2 + (l5 - l1*cos(phi_1) + l4*cos(phi_4))^2 + l2^2 - l3^2)^2 + 4*l2^2*(l5 - l1*cos(phi_1) + l4*cos(phi_4))^2)^(1/2) - 2*l2*(l1*sin(phi_1) - l4*sin(phi_4)))*(2*l2*l4*sin(phi_4) + 2*l4*cos(phi_4)*(l1*sin(phi_1) - l4*sin(phi_4)) + 2*l4*sin(phi_4)*(l5 - l1*cos(phi_1) + l4*cos(phi_4))))/((l1*sin(phi_1) - l4*sin(phi_4))^2 + (l5 - l1*cos(phi_1) + l4*cos(phi_4))^2 + l2^2 - l3^2 + 2*l2*(l5 - l1*cos(phi_1) + l4*cos(phi_4)))^2))/((((4*l2^2*(l1*sin(phi_1) - l4*sin(phi_4))^2 - ((l1*sin(phi_1) - l4*sin(phi_4))^2 + (l5 - l1*cos(phi_1) + l4*cos(phi_4))^2 + l2^2 - l3^2)^2 + 4*l2^2*(l5 - l1*cos(phi_1) + l4*cos(phi_4))^2)^(1/2) - 2*l2*(l1*sin(phi_1) - l4*sin(phi_4)))^2/((l1*sin(phi_1) - l4*sin(phi_4))^2 + (l5 - l1*cos(phi_1) + l4*cos(phi_4))^2 + l2^2 - l3^2 + 2*l2*(l5 - l1*cos(phi_1) + l4*cos(phi_4)))^2 + 1)*(l2*cos(2*atan(((4*l2^2*(l1*sin(phi_1) - l4*sin(phi_4))^2 - ((l1*sin(phi_1) - l4*sin(phi_4))^2 + (l5 - l1*cos(phi_1) + l4*cos(phi_4))^2 + l2^2 - l3^2)^2 + 4*l2^2*(l5 - l1*cos(phi_1) + l4*cos(phi_4))^2)^(1/2) - 2*l2*(l1*sin(phi_1) - l4*sin(phi_4)))/((l1*sin(phi_1) - l4*sin(phi_4))^2 + (l5 - l1*cos(phi_1) + l4*cos(phi_4))^2 + l2^2 - l3^2 + 2*l2*(l5 - l1*cos(phi_1) + l4*cos(phi_4))))) - l5/2 + l1*cos(phi_1))^2)))/((l2*sin(2*atan(((4*l2^2*(l1*sin(phi_1) - l4*sin(phi_4))^2 - ((l1*sin(phi_1) - l4*sin(phi_4))^2 + (l5 - l1*cos(phi_1) + l4*cos(phi_4))^2 + l2^2 - l3^2)^2 + 4*l2^2*(l5 - l1*cos(phi_1) + l4*cos(phi_4))^2)^(1/2) - 2*l2*(l1*sin(phi_1) - l4*sin(phi_4)))/((l1*sin(phi_1) - l4*sin(phi_4))^2 + (l5 - l1*cos(phi_1) + l4*cos(phi_4))^2 + l2^2 - l3^2 + 2*l2*(l5 - l1*cos(phi_1) + l4*cos(phi_4))))) + l1*sin(phi_1))^2/(l2*cos(2*atan(((4*l2^2*(l1*sin(phi_1) - l4*sin(phi_4))^2 - ((l1*sin(phi_1) - l4*sin(phi_4))^2 + (l5 - l1*cos(phi_1) + l4*cos(phi_4))^2 + l2^2 - l3^2)^2 + 4*l2^2*(l5 - l1*cos(phi_1) + l4*cos(phi_4))^2)^(1/2) - 2*l2*(l1*sin(phi_1) - l4*sin(phi_4)))/((l1*sin(phi_1) - l4*sin(phi_4))^2 + (l5 - l1*cos(phi_1) + l4*cos(phi_4))^2 + l2^2 - l3^2 + 2*l2*(l5 - l1*cos(phi_1) + l4*cos(phi_4))))) - l5/2 + l1*cos(phi_1))^2 + 1);
end

    % syms phi_0 phi_1 phi_2 phi_4 l1 l2 l3 l4 l5 L0 d_phi1 d_phi4
    % 
    % XD=l5+l4*cos(phi_4);
    % YD=l4*sin(phi_4);
    % XB=l1*cos(phi_1);
    % YB=l1*sin(phi_1);
    % A0=2*l2*(XD-XB);
    % B0=2*l2*(YD-YB);
    % lBD=sqrt((XD-XB)^2+(YD-YB)^2);
    % C0=l2^2+lBD^2-l3^2;
    % phi_2=2*atan((B0+sqrt(A0^2+B0^2-C0^2))/(A0+C0));
    % XC=XB+l2*cos(phi_2);
    % YC=YB+l2*sin(phi_2);
    % L0=sqrt((XC-l5/2)^2+YC^2);
    % phi_0=atan(YC/(XC-l5/2));
    % 
    % J=jacobian([L0;phi_0],[phi_1;phi_4]);
    % phi0_dot = J(2,1)*d_phi1 +J(2,2)*d_phi4

    % jacobian函数无法在simulink中使用，故直接使用jacobian函数的最终结果

== matlab function blance_leg2/Subsystem4/MATLAB Function9 ==
  data: F0 input; T1 output; Tp input; phi1 input; phi4 input; T2 output
function [T1,T2] = VMC_calc(F0,Tp,phi1,phi4)

    l5=0.08;%AE长度
    l1=0.075;
    l2=0.14;
    l3=0.14;
    l4=0.075;

YD = l4*sin(phi4);
YB = l1*sin(phi1);
XD = l5 + l4*cos(phi4);
XB = l1*cos(phi1); 
lBD = sqrt((XD - XB)*(XD - XB) + (YD - YB)*(YD - YB));
A0 = 2*l2*(XD - XB);
B0 = 2*l2*(YD - YB);
C0 = l2*l2 + lBD*lBD - l3*l3;
phi2 = 2*atan2((B0 + sqrt(A0*A0 + B0*B0 - C0*C0)),A0 + C0);
phi3 = atan2(YB-YD+l2*sin(phi2),XB-XD+l2*cos(phi2));
XC = l1*cos(phi1) + l2*cos(phi2);
YC = l1*sin(phi1) + l2*sin(phi2);
L0 = sqrt((XC - l5/2)*(XC - l5/2) + YC*YC);
phi0 = atan2(YC,XC - l5/2);
j11 = (l1*sin(phi0-phi3)*sin(phi1-phi2))/sin(phi3-phi2);
j12 = (l1*cos(phi0-phi3)*sin(phi1-phi2))/(L0*sin(phi3-phi2));
j21 = (l4*sin(phi0-phi2)*sin(phi3-phi4))/sin(phi3-phi2);
j22 = (l4*cos(phi0-phi2)*sin(phi3-phi4))/(L0*sin(phi3-phi2));
J = [j11 j12; j21 j22];
F = [F0;Tp];
T = J * F;
T1 = T(1,1);
T2 = T(2,1);
end
